simulink model "Inversor_Real_v2"  (R2026b)
settings: Solver=VariableStepAuto
values from neighbouring files (symbols this model uses):
  sat_V = sqrt(2/3)*V_slMAX    [coeficientes.m]
  wn_V = 8500    [coeficientes.m]
  zeta_V = 1    [coeficientes.m]
settings Model: Creator=fedeb  LastModifiedBy=fedeb

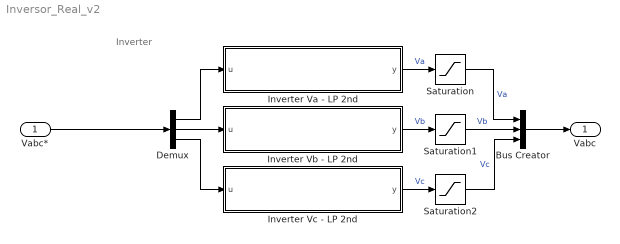
== system Inversor_Real_v2 ==
  note: Inverter
  Vabc* : Inport
  Bus Creator : BusCreator  Inputs=3
  Demux : Demux  Outputs=3
  Inverter Va - LP 2nd : Subsystem
  Inverter Vb - LP 2nd : Subsystem
  Inverter Vc - LP 2nd : Subsystem
  Saturation : Saturate  UpperLimit=sat_V  LowerLimit=-sat_V
  Saturation1 : Saturate  UpperLimit=sat_V  LowerLimit=-sat_V
  Saturation2 : Saturate  UpperLimit=sat_V  LowerLimit=-sat_V
  Vabc : Outport
  wires:
  Bus Creator/1 -> Vabc/1
  Demux/3 -> Inverter Vc - LP 2nd/1(u)
  Demux/2 -> Inverter Vb - LP 2nd/1(u)
  Demux/1 -> Inverter Va - LP 2nd/1(u)
  Saturation1/1 -> Bus Creator/2  "Vb"
  Saturation/1 -> Bus Creator/1  "Va"
  Inverter Vb - LP 2nd/1(y) -> Saturation1/1  "Vb"
  Saturation2/1 -> Bus Creator/3  "Vc"
  Inverter Va - LP 2nd/1(y) -> Saturation/1  "Va"
  Vabc*/1 -> Demux/1
  Inverter Vc - LP 2nd/1(y) -> Saturation2/1  "Vc"

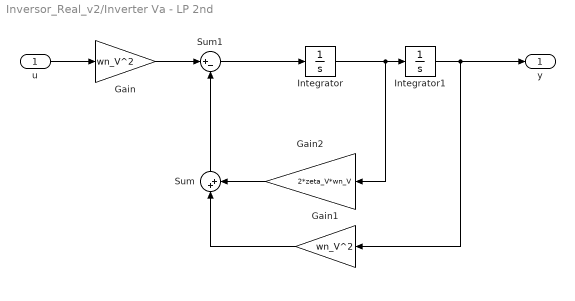
== system Inversor_Real_v2/Inverter Va - LP 2nd ==
  u : Inport
  Gain : Gain  Gain=wn_V^2
  Gain1 : Gain  Gain=wn_V^2
  Gain2 : Gain  Gain=2*zeta_V*wn_V
  Integrator : Integrator
  Integrator1 : Integrator
  Sum : Sum  Inputs=|++
  Sum1 : Sum  Inputs=|+-
  y : Outport
  wires:
  u/1 -> Gain/1
  Gain/1 -> Sum1/1
  Sum/1 -> Sum1/2
  Sum1/1 -> Integrator/1
  Gain2/1 -> Sum/2
  Gain1/1 -> Sum/1
  Integrator/1 -> Gain2/1, Integrator1/1
  Integrator1/1 -> Gain1/1, y/1

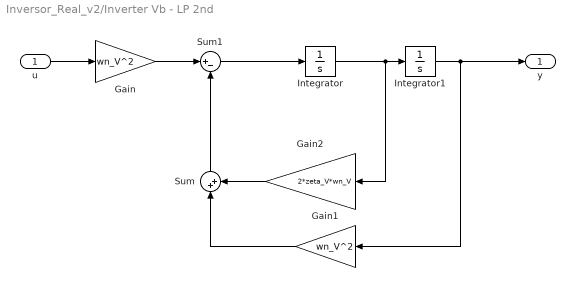
== system Inversor_Real_v2/Inverter Vb - LP 2nd ==
  u : Inport
  Gain : Gain  Gain=wn_V^2
  Gain1 : Gain  Gain=wn_V^2
  Gain2 : Gain  Gain=2*zeta_V*wn_V
  Integrator : Integrator
  Integrator1 : Integrator
  Sum : Sum  Inputs=|++
  Sum1 : Sum  Inputs=|+-
  y : Outport
  wires:
  Integrator1/1 -> y/1, Gain1/1
  Integrator/1 -> Integrator1/1, Gain2/1
  Gain1/1 -> Sum/1
  Gain2/1 -> Sum/2
  Sum1/1 -> Integrator/1
  Sum/1 -> Sum1/2
  Gain/1 -> Sum1/1
  u/1 -> Gain/1

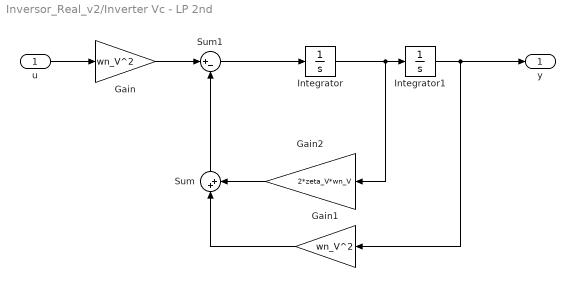
== system Inversor_Real_v2/Inverter Vc - LP 2nd ==
  u : Inport
  Gain : Gain  Gain=wn_V^2
  Gain1 : Gain  Gain=wn_V^2
  Gain2 : Gain  Gain=2*zeta_V*wn_V
  Integrator : Integrator
  Integrator1 : Integrator
  Sum : Sum  Inputs=|++
  Sum1 : Sum  Inputs=|+-
  y : Outport
  wires:
  u/1 -> Gain/1
  Gain/1 -> Sum1/1
  Sum/1 -> Sum1/2
  Sum1/1 -> Integrator/1
  Gain2/1 -> Sum/2
  Gain1/1 -> Sum/1
  Integrator/1 -> Gain2/1, Integrator1/1
  Integrator1/1 -> Gain1/1, y/1
